simulink model "QD2_DroneStack_MPC"  (R2023b)
settings: Solver=ode1  StartTime=0.0  StopTime=inf  FixedStep=1/1000  RelTol=1e-3  EnableMultiTasking=on
InitFcn:
  | % QD2_DroneStack_MPC: rutas de la librería qd2_* y del mapeo de motores
  | qd2_d = fileparts(get_param(bdroot, 'FileName'));
  | for qd2_k = 1:4
  |     if exist(fullfile(qd2_d, 'lib', 'qd2_params.m'), 'file'), break; end
  |     qd2_d = fileparts(qd2_d);
  | end
  | addpath(fullfile(qd2_d, 'lib'));
  | addpath(fullfile(qd2_d, 'equipo2_original'));
  | clear qd2_d qd2_k
  | Motor_Mapping_7_Inch
model workspace (MAT data in the model file):
  target_system = 1
undefined symbols (not defined in the file): _Commander, _QDrone2, _Stabilizer, datetime, HIL, KT, lf, log_, m, Motor_Matrix, n, qc_get_step_size, s, saved_data
libraries: quarc_library x94, simulink x27, simulink_extras x9
(part 5 of 5)

== matlab function QD2_DroneStack_MPC/HORIZON FRAME CONVERSION AND ESTIMATION/Pose Switchbox/MATLAB Function ==
  data: sigmoid_type input; enable output; x_des input; slow_lim input; fast_lim input; x_cur input; x_vel input; x_ref output; max_x_vel output; max_x_accel output; x_meas input
function [enable, x_ref, max_x_vel, max_x_accel] = fcn(sigmoid_type, x_des, slow_lim, fast_lim, x_cur, x_vel, x_meas)

% Note: Some of the cases below are identical. However, they are separated out 
% based on the states of the state machine for ease of modification in the future. 
% For example, states 4 and 5 are identical. However, if the user wants different 
% signmoid behaviour when taking off than when landing, these cases may not be the same. 

enable = 0;
x_ref = 0;
max_x_vel = 0;
max_x_accel = 0;

switch sigmoid_type
    case 1 % This is for the IDLE, ARM, E_ABORT, E_STOP and DISABLE states of the FSM
        enable = 1;
        x_ref = x_meas;
        max_x_vel = slow_lim(1);
        max_x_accel = slow_lim(2);

    case 2 % This is for the TAKEOFF THROTTLE state of the FSM
        enable = 1;
        x_ref = x_meas;
        max_x_vel = slow_lim(1);
        max_x_accel = slow_lim(2);

    case 3 % This is for the FLIGHT state of the FSM
        enable = 1;
        x_ref = x_des;
        max_x_vel = fast_lim(1);
        max_x_accel = fast_lim(2);

    case 4 % This is for the TAKEOFF HEIGHT state of the FSM
        enable = 1;
        x_ref = x_des;
        if (abs(x_cur - x_des) <= 0.02)
            max_x_vel = fast_lim(1);
            max_x_accel = fast_lim(2);
        else    
            max_x_vel = slow_lim(1);
            max_x_accel = slow_lim(2);
        end
    case 5 % This is for the AUTOLAND state of the FSM
        enable = 1;
        x_ref = x_des;
        if (abs(x_cur - x_des) <= 0.02)
            max_x_vel = fast_lim(1);
            max_x_accel = fast_lim(2);        
        else
            max_x_vel = slow_lim(1);
            max_x_accel = slow_lim(2);
        end
        
end

== matlab function QD2_DroneStack_MPC/HORIZON FRAME CONVERSION AND ESTIMATION/Pose Switchbox/MATLAB Function1 ==
  data: sigmoid_type input; enable output; y_des input; slow_lim input; fast_lim input; y_cur input; y_vel input; y_ref output; max_y_vel output; max_y_accel output; y_meas input
function [enable, y_ref, max_y_vel, max_y_accel] = fcn(sigmoid_type, y_des, slow_lim, fast_lim, y_cur, y_vel, y_meas)

% Note: Some of the cases below are identical. However, they are separated out 
% based on the states of the state machine for ease of modification in the future. 
% For example, states 4 and 5 are identical. However, if the user wants different 
% signmoid behaviour when taking off than when landing, these cases may not be the same. 

enable = 0;
y_ref = 0;
max_y_vel = 0;
max_y_accel = 0;

switch sigmoid_type
    case 1 % This is for the IDLE, ARM, E_ABORT, E_STOP and DISABLE states of the FSM
        enable = 1;
        y_ref = y_meas;
        max_y_vel = slow_lim(1);
        max_y_accel = slow_lim(2);

    case 2 % This is for the TAKEOFF THROTTLE state of the FSM
        enable = 1;
        y_ref = y_meas;
        max_y_vel = slow_lim(1);
        max_y_accel = slow_lim(2);

    case 3 % This is for the FLIGHT state of the FSM
        enable = 1;
        y_ref = y_des;
        max_y_vel = fast_lim(1);
        max_y_accel = fast_lim(2);

    case 4 % This is for the TAKEOFF HEIGHT state of the FSM
        enable = 1;
        y_ref = y_des;
        if (abs(y_cur - y_des) <= 0.02)
            max_y_vel = fast_lim(1);
            max_y_accel = fast_lim(2);
        else    
            max_y_vel = slow_lim(1);
            max_y_accel = slow_lim(2);
        end
    case 5 % This is for the AUTOLAND state of the FSM
        enable = 1;
        y_ref = y_des;
        if (abs(y_cur - y_des) <= 0.02)
            max_y_vel = fast_lim(1);
            max_y_accel = fast_lim(2);        
        else
            max_y_vel = slow_lim(1);
            max_y_accel = slow_lim(2);
        end
        
end
